simulink model "Pressure_actuationOnly_NDICheck"  (R2025a)
settings: Solver=FixedStepAuto  StartTime=0.0  StopTime=212  FixedStep=1/100  RelTol=1e-3
model workspace (MAT data in the model file):
  W1_l1 = [-0.00637147299334 -0.00624802223118 -0.00619603187657 0.00818749930186 -0.00424511993807 -0.00083745726232 -0.00833424331717 0.00697799997251 -0.00715003670843 -0.00626604831718 -0.0705428701228 0.00662881038519 ... (5376 elements, 64x84)]
  W1_l2 = [0 0 0 0 0 0 0 0 0 0 0 0 ... (5376 elements, 64x84)]
  W1_l3 = [0 0 0 0 0 0 0 0 0 0 0 0 ... (5376 elements, 64x84)]
  W2_l1 = [-0.0156497886645 0.016762621794 0.0167348569836 -0.0231262161799 0.0185108770145 -0.0187268245245 -0.014776023883 0.0177292072634 -0.013613498126 0.0173024291583 0.0215678825224 0.0115265826162 ... (2048 elements, 32x64)]
  W2_l2 = [-0.0377476122839 0.0538729387073 0.0438303187069 0.0464086258401 -0.0417546570682 0.011838804868 -0.0417271960925 0.0426008315381 -0.0444773085117 0.0424451718893 -0.040141386682 -0.0533310100989 ... (2048 elements, 32x64)]
  W2_l3 = [-0.00361323771562 0.0123768179777 0.0107080464844 0.0199177209848 -0.0177829565655 0.00824623343895 -0.00619824742788 -0.00214531281672 0.0148743772087 0.01947258566 0.00407370811971 -0.0163192085678 ... (2048 elements, 32x64)]
  W3_l1 = [0.132052254619 -0.375379893145 -0.446932223908 0.357797717849 -0.393217065478 0.411103098765 0.371578024157 -0.337760153494 0.140027914221 -0.315977756494 -0.307174196243 -0.120115030619 0.356467673567 -0.318946974358 0.347846013601 0.281310976805 0.0583875464577 0.341035187771 -0.108402639966 0.37428615262 0.272154792573 0.354610269588 0.262033437472 0.282937020119 0.37222138765 -0.345991210732 0.35357076636 -0.246019830912 -0.361246203311 0.0361489089525 0.40631829349 0.390690402431]
  W3_l2 = [0.279554184021 -0.471512064684 -0.325051298271 -0.35734053232 0.304912543396 -0.0794739072662 0.308632495485 -0.320908393214 0.332378526357 -0.310167970162 0.29099894839 0.446829975634 0.303810467191 0.477454562285 -0.287813872997 -0.0111323390057 0.193873983403 0.351262861783 0.471229802796 0.131329363324 0.252671908376 -0.266031883449 -0.00894939785395 0.202914977496 0.366234669191 -0.479416914538 -0.277658363731 -0.471064052281 -0.33223002997 0.33649823773 -0.3237987287 -0.152648432709]
  W3_l3 = [-0.0570001238091 0.199424322924 0.209089111533 0.603627643255 -0.418786165651 0.0997717774498 -0.0840156243336 -0.0236237427471 0.379327938099 0.50292362288 0.0108831688655 -0.34227191869 0.0496008214244 0.003454081698 0.42954582127 -0.0891536832515 -0.26022340414 0.0132125941854 0.620247612924 0.0666411132679 0.233222383017 -0.523892706137 0.173698824925 -0.241772112927 0.242441790042 -0.0986814410551 -0.504986125384 0.488996142317 0.327293966333 -0.125785479986 0.240581354798 -0.177036443445]
  b1_l1 = [0.00710175645196; 0.000369184720508; 0.000710181990281; 0.0393455266092; 0.00950708970836; 0.0109777156356; -0.0133124765123; -0.00522158774426; 0.00164422558321; 0.00576255868365; -0.0478743336823; -0.00160511772982; -0.00142978023771; -0.00639741085861; 0.038590241385; -0.0094911127386; 0.00815014497441; -0.00642904447059; 0.0149798978272; 0.00955784982949; -0.0605976483725; 0.103661968045; -0.00627958976617; 0.0688297117201; -0.21334497035; -0.0251886620197; -0.00479869017485; -0.000374393840524; -0.000543048749779; 0.000962840122552; 0.0269692925837; -0.00156041401416; 0.157596757208; -0.0415610568693; 0.00996469029663; 0.00986181258243; 0.00406416866301; -0.0476783919999; 0.00328716599118; 0.00912061084169; -0.0574355192967; 0.339847077609; -0.00835363476843; 0.0233594129718; -0.0202479260574; -0.0621467587317; 0.00927216812638; -0.073965203923; 0.0304471376669; -0.00934546041838; -0.00438990733048; 0.00670887951815; 0.011029799096; 0.00787045758509; 0.00135100502317; -0.00609232078954; -0.000150649756728; -0.00751443845364; -0.023495908534; -0.0060600904463; 0.0128624150416; -0.00955908948429; -0.00970156480231; -0.202157057611]
  b1_l2 = [-0.0147426613482; -0.00869580439207; 0.0138765328616; 0.0138284489813; 0.000295621534183; 0.00725342474904; -0.0162273626443; 0.0446493349263; -0.0905339713803; -0.00601908350527; 0.00965038861913; 0.0030522537524; 0.00771737097309; -0.0031772245762; -0.00467428428451; 0.199975274546; -0.00099147968196; 0.00495447699348; -0.00273156386625; 0.0198884368413; 0.000806791020795; -0.0261864850031; -0.00459526700435; 1.340144962e-05; 0.00138786673722; 0.000204867277333; -0.00857518655547; 0.00104580147611; 0.00240288575643; -0.00641972426168; -0.00170664979241; 0.0996687720208; -0.00210916748322; -0.00557769560803; -0.00795003304866; -0.19306721383; -0.000393120488751; 0.0045069662762; -0.00573219697733; 9.58917626601e-05; 0.00417395073964; 0.00562640384847; -0.00129112919515; -0.0482075402567; -0.00196858006629; 0.000270646807413; 0.00629034710254; -0.00470403583482; -0.00171635711871; -0.00785698712492; 0.000637659281956; -0.00214698935425; -0.00202759889409; -0.105682274905; -0.00371133978013; -0.00942114780261; -0.00287472180758; -0.0024803019133; -0.0054886348773; 0.0166856153903; 0.0548659368505; -0.0153805174502; 0.0168831628843; -0.00185862406939]
  b1_l3 = [-0.000999045790686; 0.000698575449992; -0.000605690473725; 0.00160280732153; 0.000523282728528; -0.00213430900699; 0.0122687697595; 0.0390874045108; -0.00278736371045; 9.98305151793e-05; -0.0103509580715; -0.00835315937259; 0.0125017612217; 0.000131003206606; -0.00355506191444; -0.00390199644968; -0.00106611990826; 0.151912741453; -0.000553834812616; 0.0200153889345; 0.00351918947547; 0.0116122983294; -0.0547304513813; -0.00179479574857; -0.0253721056482; 0.00198951617988; -0.00012220417272; -0.0251474734684; -0.00319937236274; -0.112622929657; -0.000178560720775; 0.0864355695652; -0.000865907846812; 0.016576695077; 0.0404398545254; 0.0033784439568; 0.0871312954491; -0.000807144557724; 0.0150049218379; 0.00290428199341; -0.0154659647443; 0.00827559213336; 0.0157335529794; 0.0116406253115; 0.00139521235881; -0.00307951284634; -0.0122898809711; 0.00305518519486; -0.000464881011032; 0.00608566665349; 0.000526151017129; -0.00646478018707; -0.000926902805426; 0.018192857707; 0.0740929157481; 0.00313729529832; 0.00242356883212; -0.00476205378341; 0.00384515173419; 0.00134019575164; 0.00276968818103; -0.0235390841732; -0.00102259172527; -0.00118694869674]
  b2_l1 = [-0.000401046663753; -0.00628788563213; -0.0346303888099; -0.00586372666504; -0.00699317952995; 0.0114299600793; 0.00801395570366; 9.06123695651e-06; -0.00162311128817; 0.00111045782214; 0.00577555943279; 0.00114995118652; 0.00367264656621; -0.0100904874079; -0.000709363624865; -0.00174786117122; -0.000654703219236; 0.00243849848703; 0.00044985181721; 0.00840520665554; -0.00527565330271; 0.00869180260814; -0.0038625485074; 0.000547116812718; 0.00709421863772; -0.00335165994807; 0.00306704289395; 0.00411247921667; -0.00631844695392; -0.00287237314353; 0.0117555077971; 0.00518804292966]
  b2_l2 = [-0.00687229898615; -0.0142918895776; 7.1088213054e-05; 0.000748920257724; -0.00405581737759; 0.00582158552269; -0.00525058718115; 0.000648576074579; -0.00268108657353; 0.00285048552601; -0.00419904310146; 0.00427594767426; -0.00502232862763; 0.0092622467413; 0.00483527848612; -0.000844583501019; -0.00923014450363; -0.00118033431138; 0.00710790724871; -0.00942703813736; -0.00594604412095; 0.00801846254442; 0.00186846861585; -0.00864792761222; 0.001047752816; -0.0115269127434; 0.00565506385006; -0.0104373435705; 0.00164365797684; -0.00175973518347; 0.00274788420561; 0.0074649525587]
  b2_l3 = [0.000387927607183; -0.00245267007242; 0.00370637057149; 0.0310088937782; -0.0366301531366; -0.00271870043869; 0.00169361465885; 0.000929703220207; 0.0102090594854; 0.0356739380334; -0.00594828418232; 0.000255561344574; -0.00171765513408; -0.00180365266587; 0.0358926113222; 0.00217591701788; 0.00246903482849; -0.000746126078892; 0.0264303317662; 0.00448673782558; -0.00162846151488; -0.00642600866642; 0.00284382244058; 0.00494763544897; -0.00224689682866; 0.00205438609198; -0.00430248205193; 0.00263372805239; 0.00526912588126; 0.00114819596714; -0.00155024150817; 0.0018114266701]
  b3_l1 = -0.00698359211629
  b3_l2 = -0.0434220447048
  b3_l3 = 0.00285349149877
  muX_l1 = [1.57694541084; 0; 0; -0.00336127639137; 0; 0; 0.0206891205991; 0; 0; 1.57697902361; 0; 0; -0.00759973640854; 0; 0; 0.0206891205991; 0; 0; 1.57705502097; 0; 0; -0.0118194537747; 0; 0; 0.0206891205991; 0; 0; 1.57717321551; 0; 0; -0.0160019480889; 0; 0; 0.0206891205991; 0; 0; 1.57733323499; 0; 0; -0.0201289345648; 0; 0; 0.0206891205991; 0; 0; 1.57753452434; 0; 0; -0.0241823954864; 0; 0; 0.0206891205991; 0; 0; 1.57777634829; 0; 0; -0.0281446503227; 0; 0; 0.0206891205991; 0; 0; 1.57805779479; 0; 0; -0.0319984242293; 0; 0; 0.0206891205991; 0; 0; 1.57837777904; 0; 0; -0.0361987416019; 0; 0; 0.0201873644526; 0; 0; 0.0157836834877; 0.0157827615715; 0.0157817125837]
  muX_l2 = [0; 1.57694541084; 0; 0; -0.00336127639137; 0; 0; 0.0206891205991; 0; 0; 1.57697902361; 0; 0; -0.00759973640854; 0; 0; 0.0206891205991; 0; 0; 1.57705502097; 0; 0; -0.0118194537747; 0; 0; 0.0206891205991; 0; 0; 1.57717321551; 0; 0; -0.0160019480889; 0; 0; 0.0206891205991; 0; 0; 1.57733323499; 0; 0; -0.0201289345648; 0; 0; 0.0206891205991; 0; 0; 1.57753452434; 0; 0; -0.0241823954864; 0; 0; 0.0206891205991; 0; 0; 1.57777634829; 0; 0; -0.0281446503227; 0; 0; 0.0206891205991; 0; 0; 1.57805779479; 0; 0; -0.0319984242293; 0; 0; 0.0206891205991; 0; 0; 1.57837777904; 0; 0; -0.0361987416019; 0; 0; 0.0201873644526; 0; 0.0112295690764; 0.0112287489568; 0.011227921264]
  muX_l3 = [0; 0; 1.57694541084; 0; 0; -0.00336127639137; 0; 0; 0.0206891205991; 0; 0; 1.57697902361; 0; 0; -0.00759973640854; 0; 0; 0.0206891205991; 0; 0; 1.57705502097; 0; 0; -0.0118194537747; 0; 0; 0.0206891205991; 0; 0; 1.57717321551; 0; 0; -0.0160019480889; 0; 0; 0.0206891205991; 0; 0; 1.57733323499; 0; 0; -0.0201289345648; 0; 0; 0.0206891205991; 0; 0; 1.57753452434; 0; 0; -0.0241823954864; 0; 0; 0.0206891205991; 0; 0; 1.57777634829; 0; 0; -0.0281446503227; 0; 0; 0.0206891205991; 0; 0; 1.57805779479; 0; 0; -0.0319984242293; 0; 0; 0.0206891205991; 0; 0; 1.57837777904; 0; 0; -0.0361987416019; 0; 0; 0.0201873644526; 0.0148876223547; 0.014888085085; 0.0148882347893]
  muY_l1 = 0.0157844107063
  muY_l2 = 0.0112303577139
  muY_l3 = 0.0148868176685
  sigX_l1 = [1.05565395992; 1e-08; 1e-08; 4.060486428; 1e-08; 1e-08; 0.995838667948; 1e-08; 1e-08; 1.0556525752; 1e-08; 1e-08; 4.05505390791; 1e-08; 1e-08; 0.995838667948; 1e-08; 1e-08; 1.05564570018; 1e-08; 1e-08; 4.04965740302; 1e-08; 1e-08; 0.995838667948; 1e-08; 1e-08; 1.05562920516; 1e-08; 1e-08; 4.04433961101; 1e-08; 1e-08; 0.995838667948; 1e-08; 1e-08; 1.0555990726; 1e-08; 1e-08; 4.03914200444; 1e-08; 1e-08; 0.995838667948; 1e-08; 1e-08; 1.05555146062; 1e-08; 1e-08; 4.03410417072; 1e-08; 1e-08; 0.995838667948; 1e-08; 1e-08; 1.05548276366; 1e-08; 1e-08; 4.02926317975; 1e-08; 1e-08; 0.995838667948; 1e-08; 1e-08; 1.0553896693; 1e-08; 1e-08; 4.02465298987; 1e-08; 1e-08; 0.995838667948; 1e-08; 1e-08; 1.05526921043; 1e-08; 1e-08; 4.02024447146; 1e-08; 1e-08; 0.995596888739; 1e-08; 1e-08; 0.0111519213195; 0.0111530491924; 0.0111543617528]
  sigX_l2 = [1e-08; 1.05565395992; 1e-08; 1e-08; 4.060486428; 1e-08; 1e-08; 0.995838667948; 1e-08; 1e-08; 1.0556525752; 1e-08; 1e-08; 4.05505390791; 1e-08; 1e-08; 0.995838667948; 1e-08; 1e-08; 1.05564570018; 1e-08; 1e-08; 4.04965740302; 1e-08; 1e-08; 0.995838667948; 1e-08; 1e-08; 1.05562920516; 1e-08; 1e-08; 4.04433961101; 1e-08; 1e-08; 0.995838667948; 1e-08; 1e-08; 1.0555990726; 1e-08; 1e-08; 4.03914200444; 1e-08; 1e-08; 0.995838667948; 1e-08; 1e-08; 1.05555146062; 1e-08; 1e-08; 4.03410417072; 1e-08; 1e-08; 0.995838667948; 1e-08; 1e-08; 1.05548276366; 1e-08; 1e-08; 4.02926317975; 1e-08; 1e-08; 0.995838667948; 1e-08; 1e-08; 1.0553896693; 1e-08; 1e-08; 4.02465298987; 1e-08; 1e-08; 0.995838667948; 1e-08; 1e-08; 1.05526921043; 1e-08; 1e-08; 4.02024447146; 1e-08; 1e-08; 0.995596888739; 1e-08; 0.0089552801319; 0.00895628044458; 0.00895729854095]
  sigX_l3 = [1e-08; 1e-08; 1.05565395992; 1e-08; 1e-08; 4.060486428; 1e-08; 1e-08; 0.995838667948; 1e-08; 1e-08; 1.0556525752; 1e-08; 1e-08; 4.05505390791; 1e-08; 1e-08; 0.995838667948; 1e-08; 1e-08; 1.05564570018; 1e-08; 1e-08; 4.04965740302; 1e-08; 1e-08; 0.995838667948; 1e-08; 1e-08; 1.05562920516; 1e-08; 1e-08; 4.04433961101; 1e-08; 1e-08; 0.995838667948; 1e-08; 1e-08; 1.0555990726; 1e-08; 1e-08; 4.03914200444; 1e-08; 1e-08; 0.995838667948; 1e-08; 1e-08; 1.05555146062; 1e-08; 1e-08; 4.03410417072; 1e-08; 1e-08; 0.995838667948; 1e-08; 1e-08; 1.05548276366; 1e-08; 1e-08; 4.02926317975; 1e-08; 1e-08; 0.995838667948; 1e-08; 1e-08; 1.0553896693; 1e-08; 1e-08; 4.02465298987; 1e-08; 1e-08; 0.995838667948; 1e-08; 1e-08; 1.05526921043; 1e-08; 1e-08; 4.02024447146; 1e-08; 1e-08; 0.995596888739; 0.0120997557729; 0.012099241662; 0.0120990692718]
  sigY_l1 = 0.0111510578581
  sigY_l2 = 0.00895432840902
  sigY_l3 = 0.0121006138289
undefined symbols (not defined in the file or in its folder): National_Instruments, PCI
libraries: sldrtlib x3
(part 1 of 2)
settings Model: Creator=dperera  LastModifiedBy=dperera
settings RTWCC: GPUComputeCapability=3.5

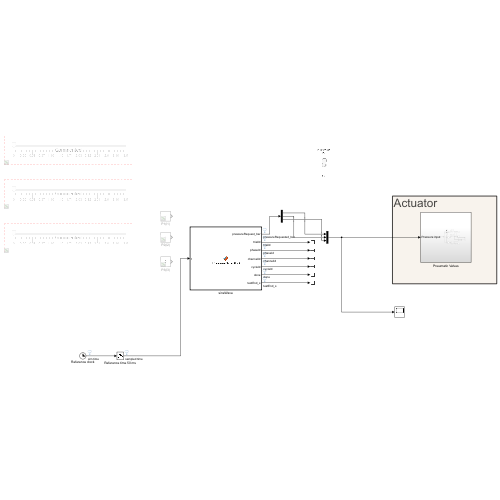
[thumbnail: Simulink's stored preview of the top-level diagram]
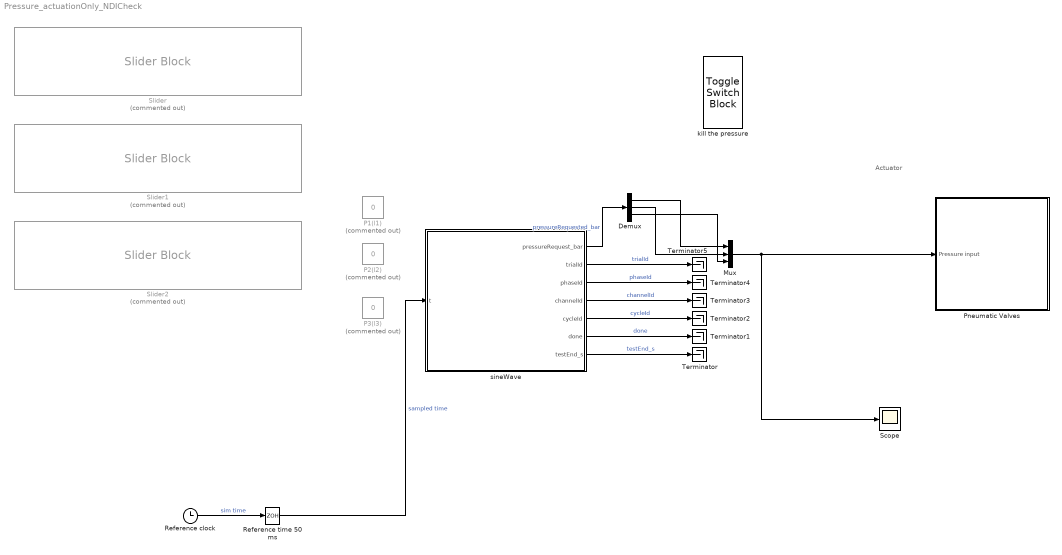
== system Pressure_actuationOnly_NDICheck ==
  note: Actuator
  Demux : Demux  Outputs=3
  Mux : Mux  Inputs=3
  P1(l1) : Constant  Commented=on  Value=0
  P2(l2) : Constant  Commented=on  Value=0
  P3(l3) : Constant  Commented=on  Value=0
  Pneumatic Valves : Subsystem
  Reference clock : Clock
  Reference time 50 ms : ZeroOrderHold  SampleTime=0.05
  Scope : Scope
      settings: ActiveDisplayYMinimum=-0.37499995347041865  ActiveDisplayYMaximum=3.3749995812337685
  Slider : SliderBlock  Commented=on  ScaleMax=3.5
  Slider1 : SliderBlock  Commented=on  ScaleMax=3.5
  Slider2 : SliderBlock  Commented=on  ScaleMax=3.5
  Terminator{,1..5} (6 alike) : Terminator
  kill the pressure : ToggleSwitchBlock
  sineWave : MATLAB Function  TreatAsAtomicUnit=on
  wires:
  Mux/1 -> Scope/1, Pneumatic Valves/1(Pressure input)
  Demux/1 -> Mux/1
  Demux/2 -> Mux/2
  Demux/3 -> Mux/3
  Reference clock/1 -> Reference time 50 ms/1  "sim time"
  Reference time 50 ms/1 -> sineWave/1(t)  "sampled time"
  sineWave/7(testEnd_s) -> Terminator/1  "testEnd_s"
  sineWave/6(done) -> Terminator1/1  "done"
  sineWave/5(cycleId) -> Terminator2/1  "cycleId"
  sineWave/4(channelId) -> Terminator3/1  "channelId"
  sineWave/3(phaseId) -> Terminator4/1  "phaseId"
  sineWave/2(trialId) -> Terminator5/1  "trialId"
  sineWave/1(pressureRequest_bar) -> Demux/1  "pressureRequested_bar"
